simulink model "SvpwmSevenSegment"  (R2026b)
settings: Solver=VariableStepAuto
settings Model: Creator=24322  LastModifiedBy=24322

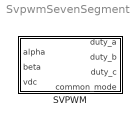
== system SvpwmSevenSegment ==
  SVPWM : Subsystem

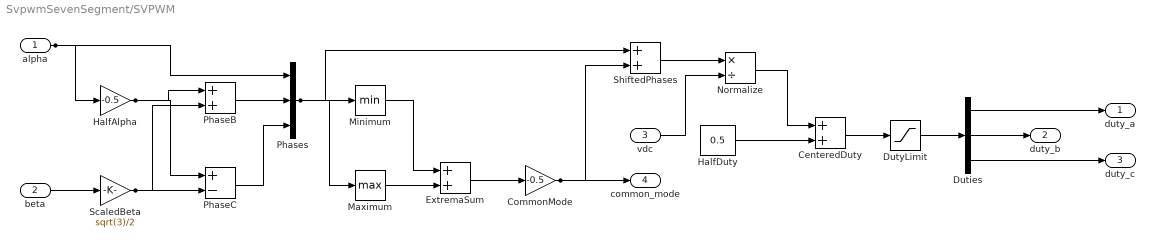
== system SvpwmSevenSegment/SVPWM ==
  alpha : Inport  OutDataTypeStr=double
  beta : Inport  Port=2  OutDataTypeStr=double
  vdc : Inport  Port=3  OutDataTypeStr=double
  CenteredDuty : Sum
  CommonMode : Gain  Gain=-0.5
  Duties : Demux  Outputs=3
  DutyLimit : Saturate  UpperLimit=1  LowerLimit=0
  ExtremaSum : Sum
  HalfAlpha : Gain  Gain=-0.5
  HalfDuty : Constant  Value=0.5
  Maximum : MinMax  Function=max
  Minimum : MinMax
  Normalize : Product  Inputs=*/
  PhaseB : Sum
  PhaseC : Sum  Inputs=+-
  Phases : Mux  Inputs=3
  ScaledBeta : Gain  Gain=sqrt(3)/2
  ShiftedPhases : Sum
  duty_a : Outport
  duty_b : Outport  Port=2
  duty_c : Outport  Port=3
  common_mode : Outport  Port=4
  wires:
  CenteredDuty/1 -> DutyLimit/1
  HalfDuty/1 -> CenteredDuty/2
  Normalize/1 -> CenteredDuty/1
  ShiftedPhases/1 -> Normalize/1
  CommonMode/1 -> ShiftedPhases/2, common_mode/1
  ExtremaSum/1 -> CommonMode/1
  Maximum/1 -> ExtremaSum/2
  Minimum/1 -> ExtremaSum/1
  Duties/3 -> duty_c/1
  Duties/2 -> duty_b/1
  Duties/1 -> duty_a/1
  DutyLimit/1 -> Duties/1
  vdc/1 -> Normalize/2
  Phases/1 -> ShiftedPhases/1, Minimum/1, Maximum/1
  PhaseC/1 -> Phases/3
  PhaseB/1 -> Phases/2
  ScaledBeta/1 -> PhaseB/2, PhaseC/2
  HalfAlpha/1 -> PhaseB/1, PhaseC/1
  beta/1 -> ScaledBeta/1
  alpha/1 -> HalfAlpha/1, Phases/1
